simulink model "Tamrin1"  (R2023b)
settings: Solver=VariableStepAuto  StartTime=0.0  StopTime=10.0  RelTol=1e-3
settings Model: Creator=hp  LastModifiedBy=hp

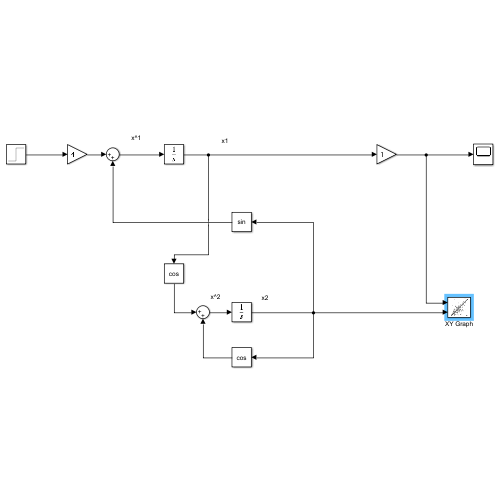
[thumbnail: Simulink's stored preview of the top-level diagram]
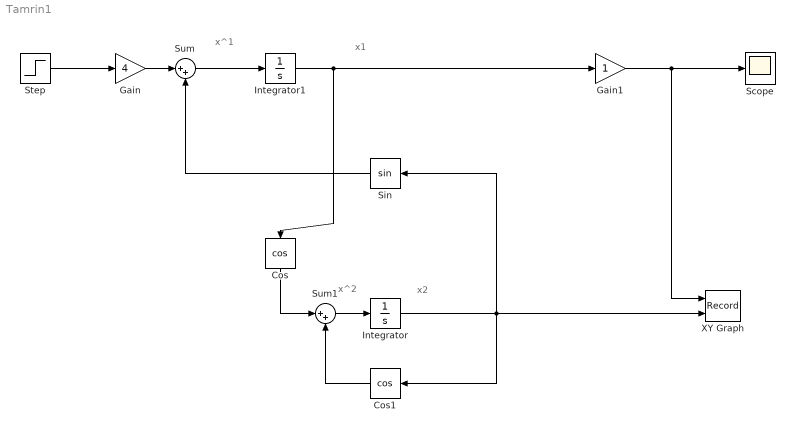
== system Tamrin1 ==
  note: x2
  note: x^2
  note: x1
  note: x^1
  Cos : Trigonometry  Operator=cos
  Cos1 : Trigonometry  Operator=cos
  Gain : Gain  Gain=4
  Gain1 : Gain
  Integrator : Integrator
  Integrator1 : Integrator
  Scope : Scope
  Sin : Trigonometry
  Step : Step  Time=0  SampleTime=0
  Sum : Sum  Inputs=|++
  Sum1 : Sum  Inputs=|++
  XY Graph : Record  FileSettingsInternal="{\"entries\":[{\"content\":{\"excelSettings\":{\"content\":{},\"type\":\"Streamout.ExcelSettings\"}},\"type\":\"Streamout.FileSettingStorage\",\"uuid\":\"\"}],\"packageUris\":[\"http:\\/\\/schema.mathworks.com\\/mf0\\/streamout_blocks\\/R2020a\"],\"version\":\"1.0\"}"  Layout=[1 1]  SignalsInternal="{\"entries\":[{\"content\":{\"signals\":[{\"content\":{\"blockPath\":[],\"dimensions\":[1],\"domain\":\"\",\"lineColor\":\"#a2142f\",\"plots\":[1],\"port\":1,\"sid\":[\"\"],\"signalID\":74,\"signalName\":\"Gain1\"},\"type\":\"RecordBlkView.Signal\",\"uuid\":\"\"},{\"content\":{\"blockPath\":[],\"dimensions\":[1],\"domain\":\"\",\"lineColor\":\"#139fff\",\"plots\":[1],\"port\":2,\"sid\":[\"\"],\"signalID\":78,\"signalName\":\"Integrator\"},\"type\":\"RecordBlkView.Signal\",\"uuid\":\"\"}]},\"type\":\"RecordBlkView.InputSignals\",\"uuid\":\"\"}],\"packageUris\":[\"http:\\/\\/schema.mathworks.com\\/mf0\\/streamout_blocks\\/R2020a\"],\"version\":\"1.0\"}"  VisualizationBindings="{\"xyplotplugin\":{\"info\":[{\"series\":[{\"bindingParametersList\":[{\"parameter\":\"X-Axis\",\"signalID\":74,\"signalName\":\"Gain1\"},{\"parameter\":\"Y-Axis\",\"signalID\":78,\"signalName\":\"Integrator\"}],\"seriesID\":39163}],\"subplotID\":1}]}}"  CompatibilityTag=XY
  wires:
  Gain/1 -> Sum/1
  Step/1 -> Gain/1
  Integrator1/1 -> Gain1/1, Cos/1
  Gain1/1 -> XY Graph/1, Scope/1
  Sum1/1 -> Integrator/1
  Cos/1 -> Sum1/1
  Cos1/1 -> Sum1/2
  Integrator/1 -> Sin/1, XY Graph/2, Cos1/1
  Sin/1 -> Sum/2
  Sum/1 -> Integrator1/1
